simulink model "DWPT_fixed"  (R2026b)
settings: Solver=ode3  StopTime=0.07  FixedStep=Ts  MaxStep=1.0E-7  RelTol=1e-4  AbsTol=1e-6
model workspace (MAT data in the model file):
  CP1 = 9.03e-09
  CP2 = 9.23e-09
  CS = 1.25e-08
  CT1 = 5.5e-08
  CT2 = 5.4e-08
  Fs = 34000000
  LP1 = 0.0004373
  LP2 = 0.0004206
  LS = 0.000306
  LT1 = 9.8e-05
  LT2 = 9.95e-05
  M1 = 9.4e-05
  M2 = 0
  RL = 30
  RP1 = 1.4
  RP2 = 1.4
  RS = 1.3
  Ts = 2.94117647059e-08
  Vdc = 50
  averageCycles = 100
  f = 85000
  samplesPerPeriod = 400
undefined symbols (not defined in the file or in its folder): ee_sli_rtmsupport, G, gcbh
libraries: sl_signal_attributes x63, eeGeneralControl x40, fl_lib x32, nesl_utility x23, eeGeneralMeasurement x14, ee_lib x9, dspfdesign x1
(part 3 of 3)

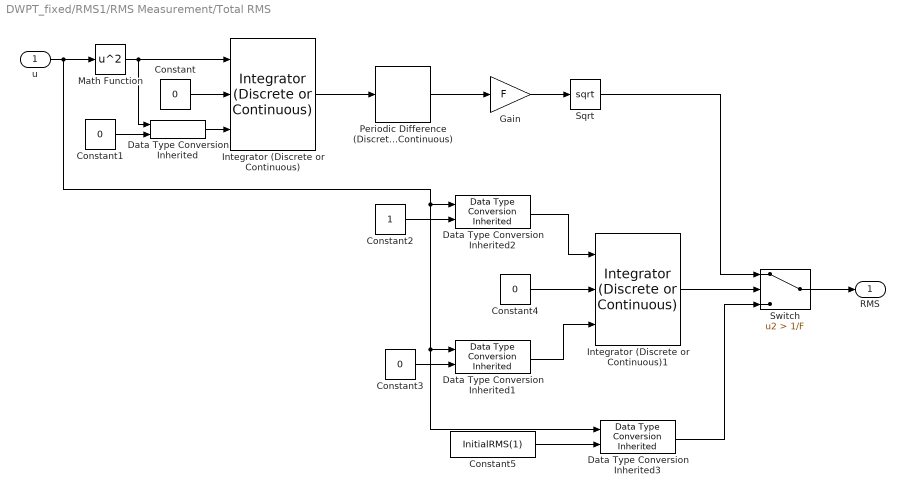
== system DWPT_fixed/RMS1/RMS Measurement/Total RMS ==
  u : Inport
  Constant{,1,3..4} (4 alike) : Constant  Value=0
  Constant2 : Constant
  Constant5 : Constant  Value=InitialRMS(1)
  Data Type Conversion Inherited{,1..3} (4 alike) : sl_signal_attributes/Data Type Conversion Inherited  ConvertRealWorld=Real World Value  DoSatur=off
  Gain : Gain  Gain=F
  Integrator (Discrete or Continuous) : eeGeneralControl/Integrator (Discrete or Continuous)  LabelModeActiveChoice=Continuous  IntegratorMethod=Integration: Forward Euler  ExternalReset=level  LimitType=Anti-windup  B=inf  A=-inf  Ts=Ts
  Integrator (Discrete or Continuous)1 : eeGeneralControl/Integrator (Discrete or Continuous)  LabelModeActiveChoice=Continuous  IntegratorMethod=Integration: Forward Euler  ExternalReset=level  LimitType=Anti-windup  B=2/F  A=-inf  Ts=Ts
  Math Function : Math  Operator=square  SignedPower=on
  Periodic Difference (Discrete or Continuous) : eeGeneralMeasurement/Periodic Difference (Discrete or Continuous)  LabelModeActiveChoice=Continuous  F=F  Ts=Ts
      link override Continuous/Transport Delay: BufferSize=262144
  Sqrt : Sqrt
  Switch : Switch  Criteria=u2 > Threshold  Threshold=1/F  SaturateOnIntegerOverflow=off  InputSameDT=off
  RMS : Outport  VectorParamsAs1DForOutWhenUnconnected=off
  wires:
  Sqrt/1 -> Switch/1
  Switch/1 -> RMS/1
  Constant2/1 -> Data Type Conversion Inherited2/2
  Constant3/1 -> Data Type Conversion Inherited1/2
  Constant4/1 -> Integrator (Discrete or Continuous)1/2
  Data Type Conversion Inherited3/1 -> Switch/3
  Constant5/1 -> Data Type Conversion Inherited3/2
  Data Type Conversion Inherited2/1 -> Integrator (Discrete or Continuous)1/1
  Data Type Conversion Inherited1/1 -> Integrator (Discrete or Continuous)1/3
  Integrator (Discrete or Continuous)1/1 -> Switch/2
  Constant1/1 -> Data Type Conversion Inherited/2
  Data Type Conversion Inherited/1 -> Integrator (Discrete or Continuous)/3
  Periodic Difference (Discrete or Continuous)/1 -> Gain/1
  Gain/1 -> Sqrt/1
  Integrator (Discrete or Continuous)/1 -> Periodic Difference (Discrete or Continuous)/1
  u/1 -> Math Function/1, Data Type Conversion Inherited2/1, Data Type Conversion Inherited3/1, Data Type Conversion Inherited1/1
  Math Function/1 -> Integrator (Discrete or Continuous)/1, Data Type Conversion Inherited/1
  Constant/1 -> Integrator (Discrete or Continuous)/2

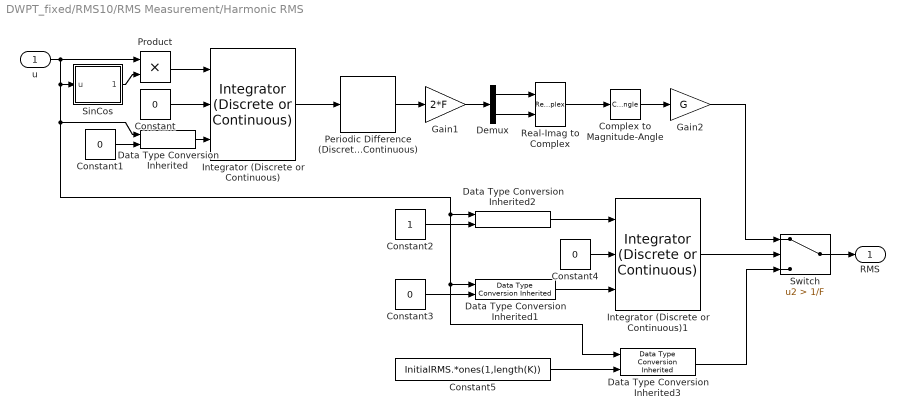
== system DWPT_fixed/RMS10/RMS Measurement/Harmonic RMS ==
  u : Inport
  Complex to Magnitude-Angle : ComplexToMagnitudeAngle  Output=Magnitude
  Constant{,1,3..4} (4 alike) : Constant  Value=0
  Constant2 : Constant
  Constant5 : Constant  Value=InitialRMS.*ones(1,length(K))
  Data Type Conversion Inherited{,1..3} (4 alike) : sl_signal_attributes/Data Type Conversion Inherited  ConvertRealWorld=Real World Value  DoSatur=off
  Demux : Demux  Outputs=2
  Gain1 : Gain  Gain=2*F
  Gain2 : Gain  Gain=G
  Integrator (Discrete or Continuous) : eeGeneralControl/Integrator (Discrete or Continuous)  LabelModeActiveChoice=Continuous  IntegratorMethod=Integration: Forward Euler  ExternalReset=level  LimitType=Anti-windup  B=inf  A=-inf  Ts=Ts
  Integrator (Discrete or Continuous)1 : eeGeneralControl/Integrator (Discrete or Continuous)  LabelModeActiveChoice=Continuous  IntegratorMethod=Integration: Forward Euler  ExternalReset=level  LimitType=Anti-windup  B=2/F  A=-inf  Ts=Ts
  Periodic Difference (Discrete or Continuous) : eeGeneralMeasurement/Periodic Difference (Discrete or Continuous)  LabelModeActiveChoice=Continuous  F=F  Ts=Ts
      link override Continuous/Transport Delay: BufferSize=262144
  Product : Product
  Real-Imag to Complex : RealImagToComplex
  SinCos : Subsystem
  Switch : Switch  Criteria=u2 > Threshold  Threshold=1/F  SaturateOnIntegerOverflow=off  InputSameDT=off
  RMS : Outport  VectorParamsAs1DForOutWhenUnconnected=off
  wires:
  Switch/1 -> RMS/1
  Gain2/1 -> Switch/1
  Constant2/1 -> Data Type Conversion Inherited2/2
  Constant3/1 -> Data Type Conversion Inherited1/2
  Constant4/1 -> Integrator (Discrete or Continuous)1/2
  Data Type Conversion Inherited3/1 -> Switch/3
  Constant5/1 -> Data Type Conversion Inherited3/2
  Data Type Conversion Inherited2/1 -> Integrator (Discrete or Continuous)1/1
  Data Type Conversion Inherited1/1 -> Integrator (Discrete or Continuous)1/3
  Integrator (Discrete or Continuous)1/1 -> Switch/2
  Constant1/1 -> Data Type Conversion Inherited/2
  Data Type Conversion Inherited/1 -> Integrator (Discrete or Continuous)/3
  Integrator (Discrete or Continuous)/1 -> Periodic Difference (Discrete or Continuous)/1
  Constant/1 -> Integrator (Discrete or Continuous)/2
  Demux/2 -> Real-Imag to Complex/2
  u/1 -> SinCos/1(u), Data Type Conversion Inherited/1, Data Type Conversion Inherited2/1, Data Type Conversion Inherited1/1, Data Type Conversion Inherited3/1, Product/1
  Periodic Difference (Discrete or Continuous)/1 -> Gain1/1
  Real-Imag to Complex/1 -> Complex to Magnitude-Angle/1
  Demux/1 -> Real-Imag to Complex/1
  SinCos/1(SinCos) -> Product/2
  Gain1/1 -> Demux/1
  Product/1 -> Integrator (Discrete or Continuous)/1
  Complex to Magnitude-Angle/1 -> Gain2/1

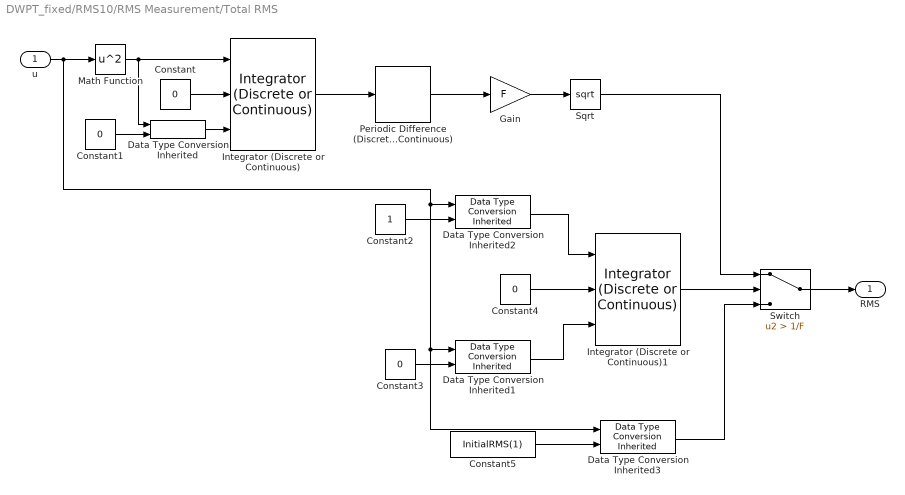
== system DWPT_fixed/RMS10/RMS Measurement/Total RMS ==
  u : Inport
  Constant{,1,3..4} (4 alike) : Constant  Value=0
  Constant2 : Constant
  Constant5 : Constant  Value=InitialRMS(1)
  Data Type Conversion Inherited{,1..3} (4 alike) : sl_signal_attributes/Data Type Conversion Inherited  ConvertRealWorld=Real World Value  DoSatur=off
  Gain : Gain  Gain=F
  Integrator (Discrete or Continuous) : eeGeneralControl/Integrator (Discrete or Continuous)  LabelModeActiveChoice=Continuous  IntegratorMethod=Integration: Forward Euler  ExternalReset=level  LimitType=Anti-windup  B=inf  A=-inf  Ts=Ts
  Integrator (Discrete or Continuous)1 : eeGeneralControl/Integrator (Discrete or Continuous)  LabelModeActiveChoice=Continuous  IntegratorMethod=Integration: Forward Euler  ExternalReset=level  LimitType=Anti-windup  B=2/F  A=-inf  Ts=Ts
  Math Function : Math  Operator=square  SignedPower=on
  Periodic Difference (Discrete or Continuous) : eeGeneralMeasurement/Periodic Difference (Discrete or Continuous)  LabelModeActiveChoice=Continuous  F=F  Ts=Ts
      link override Continuous/Transport Delay: BufferSize=262144
  Sqrt : Sqrt
  Switch : Switch  Criteria=u2 > Threshold  Threshold=1/F  SaturateOnIntegerOverflow=off  InputSameDT=off
  RMS : Outport  VectorParamsAs1DForOutWhenUnconnected=off
  wires:
  Sqrt/1 -> Switch/1
  Switch/1 -> RMS/1
  Constant2/1 -> Data Type Conversion Inherited2/2
  Constant3/1 -> Data Type Conversion Inherited1/2
  Constant4/1 -> Integrator (Discrete or Continuous)1/2
  Data Type Conversion Inherited3/1 -> Switch/3
  Constant5/1 -> Data Type Conversion Inherited3/2
  Data Type Conversion Inherited2/1 -> Integrator (Discrete or Continuous)1/1
  Data Type Conversion Inherited1/1 -> Integrator (Discrete or Continuous)1/3
  Integrator (Discrete or Continuous)1/1 -> Switch/2
  Constant1/1 -> Data Type Conversion Inherited/2
  Data Type Conversion Inherited/1 -> Integrator (Discrete or Continuous)/3
  Periodic Difference (Discrete or Continuous)/1 -> Gain/1
  Gain/1 -> Sqrt/1
  Integrator (Discrete or Continuous)/1 -> Periodic Difference (Discrete or Continuous)/1
  u/1 -> Math Function/1, Data Type Conversion Inherited2/1, Data Type Conversion Inherited3/1, Data Type Conversion Inherited1/1
  Math Function/1 -> Integrator (Discrete or Continuous)/1, Data Type Conversion Inherited/1
  Constant/1 -> Integrator (Discrete or Continuous)/2

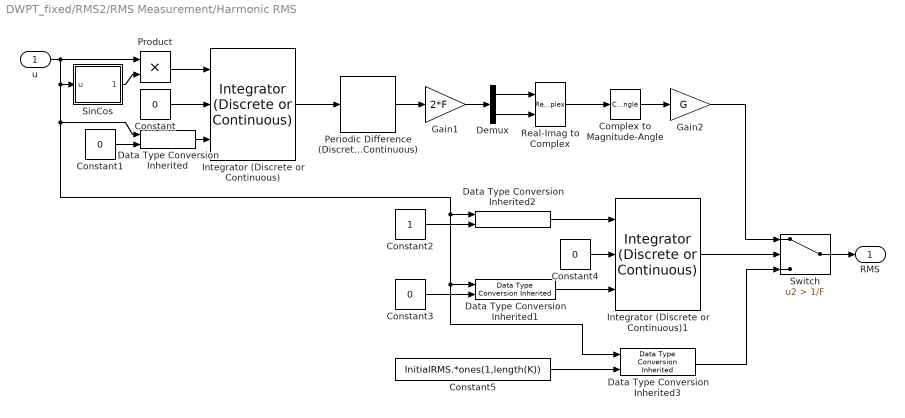
== system DWPT_fixed/RMS2/RMS Measurement/Harmonic RMS ==
  u : Inport
  Complex to Magnitude-Angle : ComplexToMagnitudeAngle  Output=Magnitude
  Constant{,1,3..4} (4 alike) : Constant  Value=0
  Constant2 : Constant
  Constant5 : Constant  Value=InitialRMS.*ones(1,length(K))
  Data Type Conversion Inherited{,1..3} (4 alike) : sl_signal_attributes/Data Type Conversion Inherited  ConvertRealWorld=Real World Value  DoSatur=off
  Demux : Demux  Outputs=2
  Gain1 : Gain  Gain=2*F
  Gain2 : Gain  Gain=G
  Integrator (Discrete or Continuous) : eeGeneralControl/Integrator (Discrete or Continuous)  LabelModeActiveChoice=Continuous  IntegratorMethod=Integration: Forward Euler  ExternalReset=level  LimitType=Anti-windup  B=inf  A=-inf  Ts=Ts
  Integrator (Discrete or Continuous)1 : eeGeneralControl/Integrator (Discrete or Continuous)  LabelModeActiveChoice=Continuous  IntegratorMethod=Integration: Forward Euler  ExternalReset=level  LimitType=Anti-windup  B=2/F  A=-inf  Ts=Ts
  Periodic Difference (Discrete or Continuous) : eeGeneralMeasurement/Periodic Difference (Discrete or Continuous)  LabelModeActiveChoice=Continuous  F=F  Ts=Ts
      link override Continuous/Transport Delay: BufferSize=262144
  Product : Product
  Real-Imag to Complex : RealImagToComplex
  SinCos : Subsystem
  Switch : Switch  Criteria=u2 > Threshold  Threshold=1/F  SaturateOnIntegerOverflow=off  InputSameDT=off
  RMS : Outport  VectorParamsAs1DForOutWhenUnconnected=off
  wires:
  Switch/1 -> RMS/1
  Gain2/1 -> Switch/1
  Constant2/1 -> Data Type Conversion Inherited2/2
  Constant3/1 -> Data Type Conversion Inherited1/2
  Constant4/1 -> Integrator (Discrete or Continuous)1/2
  Data Type Conversion Inherited3/1 -> Switch/3
  Constant5/1 -> Data Type Conversion Inherited3/2
  Data Type Conversion Inherited2/1 -> Integrator (Discrete or Continuous)1/1
  Data Type Conversion Inherited1/1 -> Integrator (Discrete or Continuous)1/3
  Integrator (Discrete or Continuous)1/1 -> Switch/2
  Constant1/1 -> Data Type Conversion Inherited/2
  Data Type Conversion Inherited/1 -> Integrator (Discrete or Continuous)/3
  Integrator (Discrete or Continuous)/1 -> Periodic Difference (Discrete or Continuous)/1
  Constant/1 -> Integrator (Discrete or Continuous)/2
  Demux/2 -> Real-Imag to Complex/2
  u/1 -> SinCos/1(u), Data Type Conversion Inherited/1, Data Type Conversion Inherited2/1, Data Type Conversion Inherited1/1, Data Type Conversion Inherited3/1, Product/1
  Periodic Difference (Discrete or Continuous)/1 -> Gain1/1
  Real-Imag to Complex/1 -> Complex to Magnitude-Angle/1
  Demux/1 -> Real-Imag to Complex/1
  SinCos/1(SinCos) -> Product/2
  Gain1/1 -> Demux/1
  Product/1 -> Integrator (Discrete or Continuous)/1
  Complex to Magnitude-Angle/1 -> Gain2/1

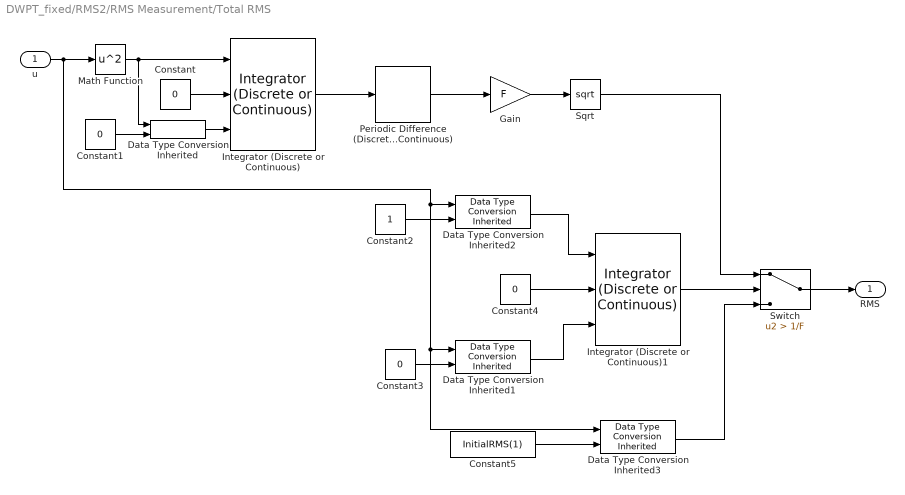
== system DWPT_fixed/RMS2/RMS Measurement/Total RMS ==
  u : Inport
  Constant{,1,3..4} (4 alike) : Constant  Value=0
  Constant2 : Constant
  Constant5 : Constant  Value=InitialRMS(1)
  Data Type Conversion Inherited{,1..3} (4 alike) : sl_signal_attributes/Data Type Conversion Inherited  ConvertRealWorld=Real World Value  DoSatur=off
  Gain : Gain  Gain=F
  Integrator (Discrete or Continuous) : eeGeneralControl/Integrator (Discrete or Continuous)  LabelModeActiveChoice=Continuous  IntegratorMethod=Integration: Forward Euler  ExternalReset=level  LimitType=Anti-windup  B=inf  A=-inf  Ts=Ts
  Integrator (Discrete or Continuous)1 : eeGeneralControl/Integrator (Discrete or Continuous)  LabelModeActiveChoice=Continuous  IntegratorMethod=Integration: Forward Euler  ExternalReset=level  LimitType=Anti-windup  B=2/F  A=-inf  Ts=Ts
  Math Function : Math  Operator=square  SignedPower=on
  Periodic Difference (Discrete or Continuous) : eeGeneralMeasurement/Periodic Difference (Discrete or Continuous)  LabelModeActiveChoice=Continuous  F=F  Ts=Ts
      link override Continuous/Transport Delay: BufferSize=262144
  Sqrt : Sqrt
  Switch : Switch  Criteria=u2 > Threshold  Threshold=1/F  SaturateOnIntegerOverflow=off  InputSameDT=off
  RMS : Outport  VectorParamsAs1DForOutWhenUnconnected=off
  wires:
  Sqrt/1 -> Switch/1
  Switch/1 -> RMS/1
  Constant2/1 -> Data Type Conversion Inherited2/2
  Constant3/1 -> Data Type Conversion Inherited1/2
  Constant4/1 -> Integrator (Discrete or Continuous)1/2
  Data Type Conversion Inherited3/1 -> Switch/3
  Constant5/1 -> Data Type Conversion Inherited3/2
  Data Type Conversion Inherited2/1 -> Integrator (Discrete or Continuous)1/1
  Data Type Conversion Inherited1/1 -> Integrator (Discrete or Continuous)1/3
  Integrator (Discrete or Continuous)1/1 -> Switch/2
  Constant1/1 -> Data Type Conversion Inherited/2
  Data Type Conversion Inherited/1 -> Integrator (Discrete or Continuous)/3
  Periodic Difference (Discrete or Continuous)/1 -> Gain/1
  Gain/1 -> Sqrt/1
  Integrator (Discrete or Continuous)/1 -> Periodic Difference (Discrete or Continuous)/1
  u/1 -> Math Function/1, Data Type Conversion Inherited2/1, Data Type Conversion Inherited3/1, Data Type Conversion Inherited1/1
  Math Function/1 -> Integrator (Discrete or Continuous)/1, Data Type Conversion Inherited/1
  Constant/1 -> Integrator (Discrete or Continuous)/2

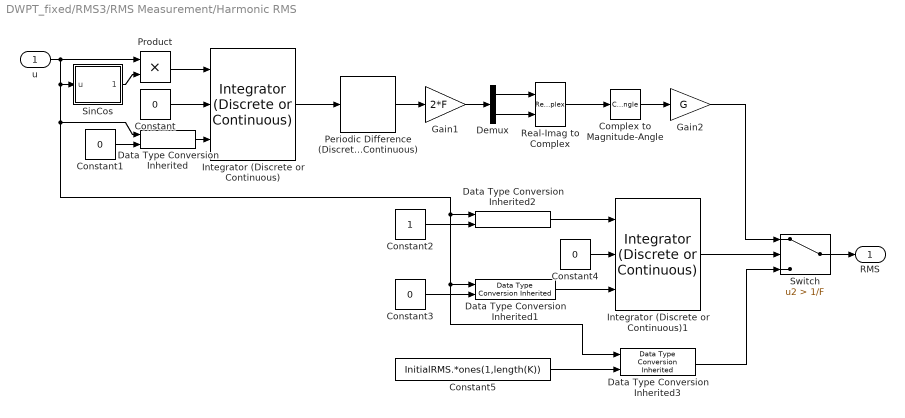
== system DWPT_fixed/RMS3/RMS Measurement/Harmonic RMS ==
  u : Inport
  Complex to Magnitude-Angle : ComplexToMagnitudeAngle  Output=Magnitude
  Constant{,1,3..4} (4 alike) : Constant  Value=0
  Constant2 : Constant
  Constant5 : Constant  Value=InitialRMS.*ones(1,length(K))
  Data Type Conversion Inherited{,1..3} (4 alike) : sl_signal_attributes/Data Type Conversion Inherited  ConvertRealWorld=Real World Value  DoSatur=off
  Demux : Demux  Outputs=2
  Gain1 : Gain  Gain=2*F
  Gain2 : Gain  Gain=G
  Integrator (Discrete or Continuous) : eeGeneralControl/Integrator (Discrete or Continuous)  LabelModeActiveChoice=Continuous  IntegratorMethod=Integration: Forward Euler  ExternalReset=level  LimitType=Anti-windup  B=inf  A=-inf  Ts=Ts
  Integrator (Discrete or Continuous)1 : eeGeneralControl/Integrator (Discrete or Continuous)  LabelModeActiveChoice=Continuous  IntegratorMethod=Integration: Forward Euler  ExternalReset=level  LimitType=Anti-windup  B=2/F  A=-inf  Ts=Ts
  Periodic Difference (Discrete or Continuous) : eeGeneralMeasurement/Periodic Difference (Discrete or Continuous)  LabelModeActiveChoice=Continuous  F=F  Ts=Ts
      link override Continuous/Transport Delay: BufferSize=262144
  Product : Product
  Real-Imag to Complex : RealImagToComplex
  SinCos : Subsystem
  Switch : Switch  Criteria=u2 > Threshold  Threshold=1/F  SaturateOnIntegerOverflow=off  InputSameDT=off
  RMS : Outport  VectorParamsAs1DForOutWhenUnconnected=off
  wires:
  Switch/1 -> RMS/1
  Gain2/1 -> Switch/1
  Constant2/1 -> Data Type Conversion Inherited2/2
  Constant3/1 -> Data Type Conversion Inherited1/2
  Constant4/1 -> Integrator (Discrete or Continuous)1/2
  Data Type Conversion Inherited3/1 -> Switch/3
  Constant5/1 -> Data Type Conversion Inherited3/2
  Data Type Conversion Inherited2/1 -> Integrator (Discrete or Continuous)1/1
  Data Type Conversion Inherited1/1 -> Integrator (Discrete or Continuous)1/3
  Integrator (Discrete or Continuous)1/1 -> Switch/2
  Constant1/1 -> Data Type Conversion Inherited/2
  Data Type Conversion Inherited/1 -> Integrator (Discrete or Continuous)/3
  Integrator (Discrete or Continuous)/1 -> Periodic Difference (Discrete or Continuous)/1
  Constant/1 -> Integrator (Discrete or Continuous)/2
  Demux/2 -> Real-Imag to Complex/2
  u/1 -> SinCos/1(u), Data Type Conversion Inherited/1, Data Type Conversion Inherited2/1, Data Type Conversion Inherited1/1, Data Type Conversion Inherited3/1, Product/1
  Periodic Difference (Discrete or Continuous)/1 -> Gain1/1
  Real-Imag to Complex/1 -> Complex to Magnitude-Angle/1
  Demux/1 -> Real-Imag to Complex/1
  SinCos/1(SinCos) -> Product/2
  Gain1/1 -> Demux/1
  Product/1 -> Integrator (Discrete or Continuous)/1
  Complex to Magnitude-Angle/1 -> Gain2/1

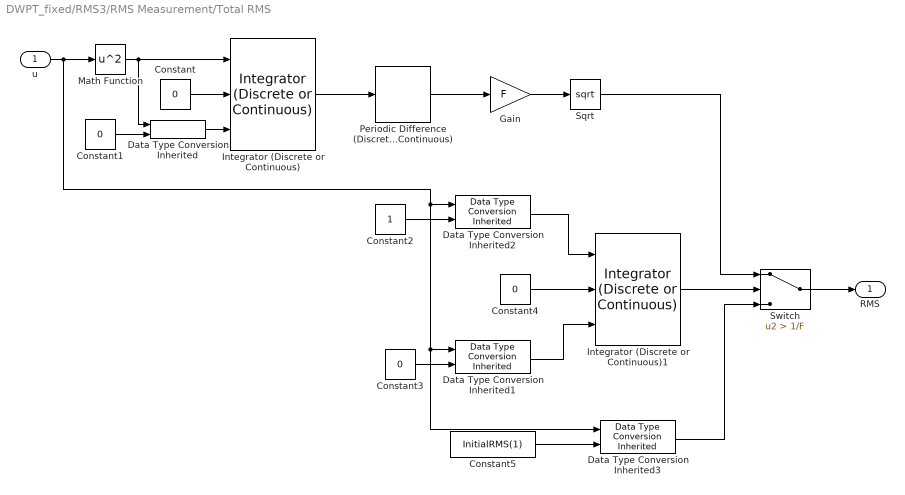
== system DWPT_fixed/RMS3/RMS Measurement/Total RMS ==
  u : Inport
  Constant{,1,3..4} (4 alike) : Constant  Value=0
  Constant2 : Constant
  Constant5 : Constant  Value=InitialRMS(1)
  Data Type Conversion Inherited{,1..3} (4 alike) : sl_signal_attributes/Data Type Conversion Inherited  ConvertRealWorld=Real World Value  DoSatur=off
  Gain : Gain  Gain=F
  Integrator (Discrete or Continuous) : eeGeneralControl/Integrator (Discrete or Continuous)  LabelModeActiveChoice=Continuous  IntegratorMethod=Integration: Forward Euler  ExternalReset=level  LimitType=Anti-windup  B=inf  A=-inf  Ts=Ts
  Integrator (Discrete or Continuous)1 : eeGeneralControl/Integrator (Discrete or Continuous)  LabelModeActiveChoice=Continuous  IntegratorMethod=Integration: Forward Euler  ExternalReset=level  LimitType=Anti-windup  B=2/F  A=-inf  Ts=Ts
  Math Function : Math  Operator=square  SignedPower=on
  Periodic Difference (Discrete or Continuous) : eeGeneralMeasurement/Periodic Difference (Discrete or Continuous)  LabelModeActiveChoice=Continuous  F=F  Ts=Ts
      link override Continuous/Transport Delay: BufferSize=262144
  Sqrt : Sqrt
  Switch : Switch  Criteria=u2 > Threshold  Threshold=1/F  SaturateOnIntegerOverflow=off  InputSameDT=off
  RMS : Outport  VectorParamsAs1DForOutWhenUnconnected=off
  wires:
  Sqrt/1 -> Switch/1
  Switch/1 -> RMS/1
  Constant2/1 -> Data Type Conversion Inherited2/2
  Constant3/1 -> Data Type Conversion Inherited1/2
  Constant4/1 -> Integrator (Discrete or Continuous)1/2
  Data Type Conversion Inherited3/1 -> Switch/3
  Constant5/1 -> Data Type Conversion Inherited3/2
  Data Type Conversion Inherited2/1 -> Integrator (Discrete or Continuous)1/1
  Data Type Conversion Inherited1/1 -> Integrator (Discrete or Continuous)1/3
  Integrator (Discrete or Continuous)1/1 -> Switch/2
  Constant1/1 -> Data Type Conversion Inherited/2
  Data Type Conversion Inherited/1 -> Integrator (Discrete or Continuous)/3
  Periodic Difference (Discrete or Continuous)/1 -> Gain/1
  Gain/1 -> Sqrt/1
  Integrator (Discrete or Continuous)/1 -> Periodic Difference (Discrete or Continuous)/1
  u/1 -> Math Function/1, Data Type Conversion Inherited2/1, Data Type Conversion Inherited3/1, Data Type Conversion Inherited1/1
  Math Function/1 -> Integrator (Discrete or Continuous)/1, Data Type Conversion Inherited/1
  Constant/1 -> Integrator (Discrete or Continuous)/2

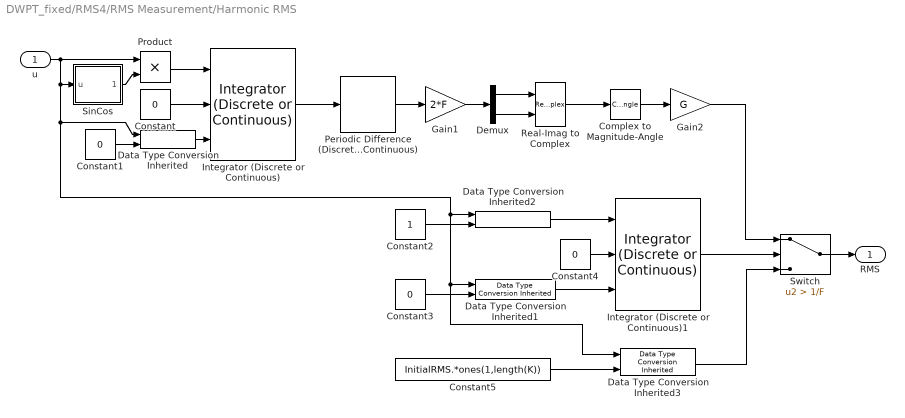
== system DWPT_fixed/RMS4/RMS Measurement/Harmonic RMS ==
  u : Inport
  Complex to Magnitude-Angle : ComplexToMagnitudeAngle  Output=Magnitude
  Constant{,1,3..4} (4 alike) : Constant  Value=0
  Constant2 : Constant
  Constant5 : Constant  Value=InitialRMS.*ones(1,length(K))
  Data Type Conversion Inherited{,1..3} (4 alike) : sl_signal_attributes/Data Type Conversion Inherited  ConvertRealWorld=Real World Value  DoSatur=off
  Demux : Demux  Outputs=2
  Gain1 : Gain  Gain=2*F
  Gain2 : Gain  Gain=G
  Integrator (Discrete or Continuous) : eeGeneralControl/Integrator (Discrete or Continuous)  LabelModeActiveChoice=Continuous  IntegratorMethod=Integration: Forward Euler  ExternalReset=level  LimitType=Anti-windup  B=inf  A=-inf  Ts=Ts
  Integrator (Discrete or Continuous)1 : eeGeneralControl/Integrator (Discrete or Continuous)  LabelModeActiveChoice=Continuous  IntegratorMethod=Integration: Forward Euler  ExternalReset=level  LimitType=Anti-windup  B=2/F  A=-inf  Ts=Ts
  Periodic Difference (Discrete or Continuous) : eeGeneralMeasurement/Periodic Difference (Discrete or Continuous)  LabelModeActiveChoice=Continuous  F=F  Ts=Ts
      link override Continuous/Transport Delay: BufferSize=262144
  Product : Product
  Real-Imag to Complex : RealImagToComplex
  SinCos : Subsystem
  Switch : Switch  Criteria=u2 > Threshold  Threshold=1/F  SaturateOnIntegerOverflow=off  InputSameDT=off
  RMS : Outport  VectorParamsAs1DForOutWhenUnconnected=off
  wires:
  Switch/1 -> RMS/1
  Gain2/1 -> Switch/1
  Constant2/1 -> Data Type Conversion Inherited2/2
  Constant3/1 -> Data Type Conversion Inherited1/2
  Constant4/1 -> Integrator (Discrete or Continuous)1/2
  Data Type Conversion Inherited3/1 -> Switch/3
  Constant5/1 -> Data Type Conversion Inherited3/2
  Data Type Conversion Inherited2/1 -> Integrator (Discrete or Continuous)1/1
  Data Type Conversion Inherited1/1 -> Integrator (Discrete or Continuous)1/3
  Integrator (Discrete or Continuous)1/1 -> Switch/2
  Constant1/1 -> Data Type Conversion Inherited/2
  Data Type Conversion Inherited/1 -> Integrator (Discrete or Continuous)/3
  Integrator (Discrete or Continuous)/1 -> Periodic Difference (Discrete or Continuous)/1
  Constant/1 -> Integrator (Discrete or Continuous)/2
  Demux/2 -> Real-Imag to Complex/2
  u/1 -> SinCos/1(u), Data Type Conversion Inherited/1, Data Type Conversion Inherited2/1, Data Type Conversion Inherited1/1, Data Type Conversion Inherited3/1, Product/1
  Periodic Difference (Discrete or Continuous)/1 -> Gain1/1
  Real-Imag to Complex/1 -> Complex to Magnitude-Angle/1
  Demux/1 -> Real-Imag to Complex/1
  SinCos/1(SinCos) -> Product/2
  Gain1/1 -> Demux/1
  Product/1 -> Integrator (Discrete or Continuous)/1
  Complex to Magnitude-Angle/1 -> Gain2/1

== system DWPT_fixed/RMS4/RMS Measurement/Total RMS ==
  u : Inport
  Constant{,1,3..4} (4 alike) : Constant  Value=0
  Constant2 : Constant
  Constant5 : Constant  Value=InitialRMS(1)
  Data Type Conversion Inherited{,1..3} (4 alike) : sl_signal_attributes/Data Type Conversion Inherited  ConvertRealWorld=Real World Value  DoSatur=off
  Gain : Gain  Gain=F
  Integrator (Discrete or Continuous) : eeGeneralControl/Integrator (Discrete or Continuous)  LabelModeActiveChoice=Continuous  IntegratorMethod=Integration: Forward Euler  ExternalReset=level  LimitType=Anti-windup  B=inf  A=-inf  Ts=Ts
  Integrator (Discrete or Continuous)1 : eeGeneralControl/Integrator (Discrete or Continuous)  LabelModeActiveChoice=Continuous  IntegratorMethod=Integration: Forward Euler  ExternalReset=level  LimitType=Anti-windup  B=2/F  A=-inf  Ts=Ts
  Math Function : Math  Operator=square  SignedPower=on
  Periodic Difference (Discrete or Continuous) : eeGeneralMeasurement/Periodic Difference (Discrete or Continuous)  LabelModeActiveChoice=Continuous  F=F  Ts=Ts
      link override Continuous/Transport Delay: BufferSize=262144
  Sqrt : Sqrt
  Switch : Switch  Criteria=u2 > Threshold  Threshold=1/F  SaturateOnIntegerOverflow=off  InputSameDT=off
  RMS : Outport  VectorParamsAs1DForOutWhenUnconnected=off
  wires:
  Sqrt/1 -> Switch/1
  Switch/1 -> RMS/1
  Constant2/1 -> Data Type Conversion Inherited2/2
  Constant3/1 -> Data Type Conversion Inherited1/2
  Constant4/1 -> Integrator (Discrete or Continuous)1/2
  Data Type Conversion Inherited3/1 -> Switch/3
  Constant5/1 -> Data Type Conversion Inherited3/2
  Data Type Conversion Inherited2/1 -> Integrator (Discrete or Continuous)1/1
  Data Type Conversion Inherited1/1 -> Integrator (Discrete or Continuous)1/3
  Integrator (Discrete or Continuous)1/1 -> Switch/2
  Constant1/1 -> Data Type Conversion Inherited/2
  Data Type Conversion Inherited/1 -> Integrator (Discrete or Continuous)/3
  Periodic Difference (Discrete or Continuous)/1 -> Gain/1
  Gain/1 -> Sqrt/1
  Integrator (Discrete or Continuous)/1 -> Periodic Difference (Discrete or Continuous)/1
  u/1 -> Math Function/1, Data Type Conversion Inherited2/1, Data Type Conversion Inherited3/1, Data Type Conversion Inherited1/1
  Math Function/1 -> Integrator (Discrete or Continuous)/1, Data Type Conversion Inherited/1
  Constant/1 -> Integrator (Discrete or Continuous)/2

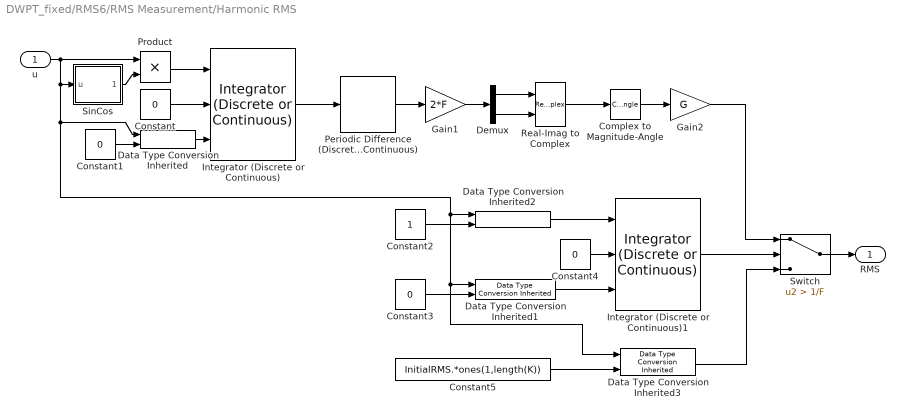
== system DWPT_fixed/RMS6/RMS Measurement/Harmonic RMS ==
  u : Inport
  Complex to Magnitude-Angle : ComplexToMagnitudeAngle  Output=Magnitude
  Constant{,1,3..4} (4 alike) : Constant  Value=0
  Constant2 : Constant
  Constant5 : Constant  Value=InitialRMS.*ones(1,length(K))
  Data Type Conversion Inherited{,1..3} (4 alike) : sl_signal_attributes/Data Type Conversion Inherited  ConvertRealWorld=Real World Value  DoSatur=off
  Demux : Demux  Outputs=2
  Gain1 : Gain  Gain=2*F
  Gain2 : Gain  Gain=G
  Integrator (Discrete or Continuous) : eeGeneralControl/Integrator (Discrete or Continuous)  LabelModeActiveChoice=Continuous  IntegratorMethod=Integration: Forward Euler  ExternalReset=level  LimitType=Anti-windup  B=inf  A=-inf  Ts=Ts
  Integrator (Discrete or Continuous)1 : eeGeneralControl/Integrator (Discrete or Continuous)  LabelModeActiveChoice=Continuous  IntegratorMethod=Integration: Forward Euler  ExternalReset=level  LimitType=Anti-windup  B=2/F  A=-inf  Ts=Ts
  Periodic Difference (Discrete or Continuous) : eeGeneralMeasurement/Periodic Difference (Discrete or Continuous)  LabelModeActiveChoice=Continuous  F=F  Ts=Ts
      link override Continuous/Transport Delay: BufferSize=262144
  Product : Product
  Real-Imag to Complex : RealImagToComplex
  SinCos : Subsystem
  Switch : Switch  Criteria=u2 > Threshold  Threshold=1/F  SaturateOnIntegerOverflow=off  InputSameDT=off
  RMS : Outport  VectorParamsAs1DForOutWhenUnconnected=off
  wires:
  Switch/1 -> RMS/1
  Gain2/1 -> Switch/1
  Constant2/1 -> Data Type Conversion Inherited2/2
  Constant3/1 -> Data Type Conversion Inherited1/2
  Constant4/1 -> Integrator (Discrete or Continuous)1/2
  Data Type Conversion Inherited3/1 -> Switch/3
  Constant5/1 -> Data Type Conversion Inherited3/2
  Data Type Conversion Inherited2/1 -> Integrator (Discrete or Continuous)1/1
  Data Type Conversion Inherited1/1 -> Integrator (Discrete or Continuous)1/3
  Integrator (Discrete or Continuous)1/1 -> Switch/2
  Constant1/1 -> Data Type Conversion Inherited/2
  Data Type Conversion Inherited/1 -> Integrator (Discrete or Continuous)/3
  Integrator (Discrete or Continuous)/1 -> Periodic Difference (Discrete or Continuous)/1
  Constant/1 -> Integrator (Discrete or Continuous)/2
  Demux/2 -> Real-Imag to Complex/2
  u/1 -> SinCos/1(u), Data Type Conversion Inherited/1, Data Type Conversion Inherited2/1, Data Type Conversion Inherited1/1, Data Type Conversion Inherited3/1, Product/1
  Periodic Difference (Discrete or Continuous)/1 -> Gain1/1
  Real-Imag to Complex/1 -> Complex to Magnitude-Angle/1
  Demux/1 -> Real-Imag to Complex/1
  SinCos/1(SinCos) -> Product/2
  Gain1/1 -> Demux/1
  Product/1 -> Integrator (Discrete or Continuous)/1
  Complex to Magnitude-Angle/1 -> Gain2/1

== system DWPT_fixed/RMS6/RMS Measurement/Total RMS ==
  u : Inport
  Constant{,1,3..4} (4 alike) : Constant  Value=0
  Constant2 : Constant
  Constant5 : Constant  Value=InitialRMS(1)
  Data Type Conversion Inherited{,1..3} (4 alike) : sl_signal_attributes/Data Type Conversion Inherited  ConvertRealWorld=Real World Value  DoSatur=off
  Gain : Gain  Gain=F
  Integrator (Discrete or Continuous) : eeGeneralControl/Integrator (Discrete or Continuous)  LabelModeActiveChoice=Continuous  IntegratorMethod=Integration: Forward Euler  ExternalReset=level  LimitType=Anti-windup  B=inf  A=-inf  Ts=Ts
  Integrator (Discrete or Continuous)1 : eeGeneralControl/Integrator (Discrete or Continuous)  LabelModeActiveChoice=Continuous  IntegratorMethod=Integration: Forward Euler  ExternalReset=level  LimitType=Anti-windup  B=2/F  A=-inf  Ts=Ts
  Math Function : Math  Operator=square  SignedPower=on
  Periodic Difference (Discrete or Continuous) : eeGeneralMeasurement/Periodic Difference (Discrete or Continuous)  LabelModeActiveChoice=Continuous  F=F  Ts=Ts
      link override Continuous/Transport Delay: BufferSize=262144
  Sqrt : Sqrt
  Switch : Switch  Criteria=u2 > Threshold  Threshold=1/F  SaturateOnIntegerOverflow=off  InputSameDT=off
  RMS : Outport  VectorParamsAs1DForOutWhenUnconnected=off
  wires:
  Sqrt/1 -> Switch/1
  Switch/1 -> RMS/1
  Constant2/1 -> Data Type Conversion Inherited2/2
  Constant3/1 -> Data Type Conversion Inherited1/2
  Constant4/1 -> Integrator (Discrete or Continuous)1/2
  Data Type Conversion Inherited3/1 -> Switch/3
  Constant5/1 -> Data Type Conversion Inherited3/2
  Data Type Conversion Inherited2/1 -> Integrator (Discrete or Continuous)1/1
  Data Type Conversion Inherited1/1 -> Integrator (Discrete or Continuous)1/3
  Integrator (Discrete or Continuous)1/1 -> Switch/2
  Constant1/1 -> Data Type Conversion Inherited/2
  Data Type Conversion Inherited/1 -> Integrator (Discrete or Continuous)/3
  Periodic Difference (Discrete or Continuous)/1 -> Gain/1
  Gain/1 -> Sqrt/1
  Integrator (Discrete or Continuous)/1 -> Periodic Difference (Discrete or Continuous)/1
  u/1 -> Math Function/1, Data Type Conversion Inherited2/1, Data Type Conversion Inherited3/1, Data Type Conversion Inherited1/1
  Math Function/1 -> Integrator (Discrete or Continuous)/1, Data Type Conversion Inherited/1
  Constant/1 -> Integrator (Discrete or Continuous)/2

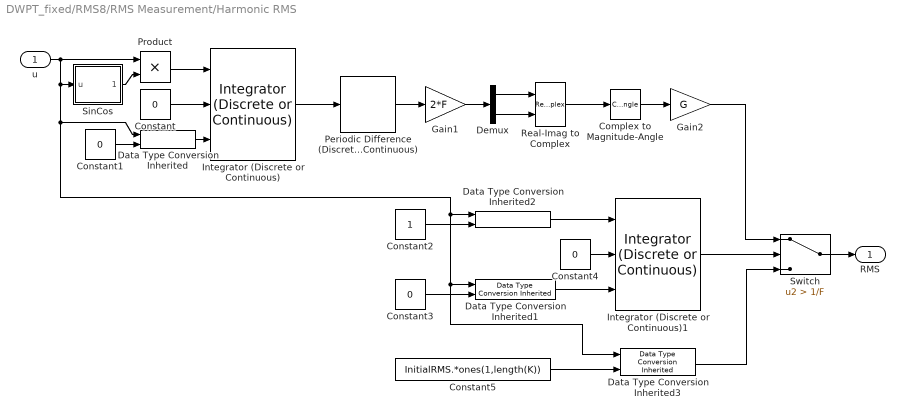
== system DWPT_fixed/RMS8/RMS Measurement/Harmonic RMS ==
  u : Inport
  Complex to Magnitude-Angle : ComplexToMagnitudeAngle  Output=Magnitude
  Constant{,1,3..4} (4 alike) : Constant  Value=0
  Constant2 : Constant
  Constant5 : Constant  Value=InitialRMS.*ones(1,length(K))
  Data Type Conversion Inherited{,1..3} (4 alike) : sl_signal_attributes/Data Type Conversion Inherited  ConvertRealWorld=Real World Value  DoSatur=off
  Demux : Demux  Outputs=2
  Gain1 : Gain  Gain=2*F
  Gain2 : Gain  Gain=G
  Integrator (Discrete or Continuous) : eeGeneralControl/Integrator (Discrete or Continuous)  LabelModeActiveChoice=Continuous  IntegratorMethod=Integration: Forward Euler  ExternalReset=level  LimitType=Anti-windup  B=inf  A=-inf  Ts=Ts
  Integrator (Discrete or Continuous)1 : eeGeneralControl/Integrator (Discrete or Continuous)  LabelModeActiveChoice=Continuous  IntegratorMethod=Integration: Forward Euler  ExternalReset=level  LimitType=Anti-windup  B=2/F  A=-inf  Ts=Ts
  Periodic Difference (Discrete or Continuous) : eeGeneralMeasurement/Periodic Difference (Discrete or Continuous)  LabelModeActiveChoice=Continuous  F=F  Ts=Ts
      link override Continuous/Transport Delay: BufferSize=262144
  Product : Product
  Real-Imag to Complex : RealImagToComplex
  SinCos : Subsystem
  Switch : Switch  Criteria=u2 > Threshold  Threshold=1/F  SaturateOnIntegerOverflow=off  InputSameDT=off
  RMS : Outport  VectorParamsAs1DForOutWhenUnconnected=off
  wires:
  Switch/1 -> RMS/1
  Gain2/1 -> Switch/1
  Constant2/1 -> Data Type Conversion Inherited2/2
  Constant3/1 -> Data Type Conversion Inherited1/2
  Constant4/1 -> Integrator (Discrete or Continuous)1/2
  Data Type Conversion Inherited3/1 -> Switch/3
  Constant5/1 -> Data Type Conversion Inherited3/2
  Data Type Conversion Inherited2/1 -> Integrator (Discrete or Continuous)1/1
  Data Type Conversion Inherited1/1 -> Integrator (Discrete or Continuous)1/3
  Integrator (Discrete or Continuous)1/1 -> Switch/2
  Constant1/1 -> Data Type Conversion Inherited/2
  Data Type Conversion Inherited/1 -> Integrator (Discrete or Continuous)/3
  Integrator (Discrete or Continuous)/1 -> Periodic Difference (Discrete or Continuous)/1
  Constant/1 -> Integrator (Discrete or Continuous)/2
  Demux/2 -> Real-Imag to Complex/2
  u/1 -> SinCos/1(u), Data Type Conversion Inherited/1, Data Type Conversion Inherited2/1, Data Type Conversion Inherited1/1, Data Type Conversion Inherited3/1, Product/1
  Periodic Difference (Discrete or Continuous)/1 -> Gain1/1
  Real-Imag to Complex/1 -> Complex to Magnitude-Angle/1
  Demux/1 -> Real-Imag to Complex/1
  SinCos/1(SinCos) -> Product/2
  Gain1/1 -> Demux/1
  Product/1 -> Integrator (Discrete or Continuous)/1
  Complex to Magnitude-Angle/1 -> Gain2/1

== system DWPT_fixed/RMS8/RMS Measurement/Total RMS ==
  u : Inport
  Constant{,1,3..4} (4 alike) : Constant  Value=0
  Constant2 : Constant
  Constant5 : Constant  Value=InitialRMS(1)
  Data Type Conversion Inherited{,1..3} (4 alike) : sl_signal_attributes/Data Type Conversion Inherited  ConvertRealWorld=Real World Value  DoSatur=off
  Gain : Gain  Gain=F
  Integrator (Discrete or Continuous) : eeGeneralControl/Integrator (Discrete or Continuous)  LabelModeActiveChoice=Continuous  IntegratorMethod=Integration: Forward Euler  ExternalReset=level  LimitType=Anti-windup  B=inf  A=-inf  Ts=Ts
  Integrator (Discrete or Continuous)1 : eeGeneralControl/Integrator (Discrete or Continuous)  LabelModeActiveChoice=Continuous  IntegratorMethod=Integration: Forward Euler  ExternalReset=level  LimitType=Anti-windup  B=2/F  A=-inf  Ts=Ts
  Math Function : Math  Operator=square  SignedPower=on
  Periodic Difference (Discrete or Continuous) : eeGeneralMeasurement/Periodic Difference (Discrete or Continuous)  LabelModeActiveChoice=Continuous  F=F  Ts=Ts
      link override Continuous/Transport Delay: BufferSize=262144
  Sqrt : Sqrt
  Switch : Switch  Criteria=u2 > Threshold  Threshold=1/F  SaturateOnIntegerOverflow=off  InputSameDT=off
  RMS : Outport  VectorParamsAs1DForOutWhenUnconnected=off
  wires:
  Sqrt/1 -> Switch/1
  Switch/1 -> RMS/1
  Constant2/1 -> Data Type Conversion Inherited2/2
  Constant3/1 -> Data Type Conversion Inherited1/2
  Constant4/1 -> Integrator (Discrete or Continuous)1/2
  Data Type Conversion Inherited3/1 -> Switch/3
  Constant5/1 -> Data Type Conversion Inherited3/2
  Data Type Conversion Inherited2/1 -> Integrator (Discrete or Continuous)1/1
  Data Type Conversion Inherited1/1 -> Integrator (Discrete or Continuous)1/3
  Integrator (Discrete or Continuous)1/1 -> Switch/2
  Constant1/1 -> Data Type Conversion Inherited/2
  Data Type Conversion Inherited/1 -> Integrator (Discrete or Continuous)/3
  Periodic Difference (Discrete or Continuous)/1 -> Gain/1
  Gain/1 -> Sqrt/1
  Integrator (Discrete or Continuous)/1 -> Periodic Difference (Discrete or Continuous)/1
  u/1 -> Math Function/1, Data Type Conversion Inherited2/1, Data Type Conversion Inherited3/1, Data Type Conversion Inherited1/1
  Math Function/1 -> Integrator (Discrete or Continuous)/1, Data Type Conversion Inherited/1
  Constant/1 -> Integrator (Discrete or Continuous)/2

== system DWPT_fixed/RMS1/RMS Measurement/Harmonic RMS/SinCos ==
  u : Inport
  Data Type Conversion Inherited : sl_signal_attributes/Data Type Conversion Inherited  ConvertRealWorld=Real World Value  DoSatur=off
  Integrator with Wrapped State (Discrete or Continuous) : eeGeneralControl/Integrator with Wrapped State (Discrete or Continuous)  LabelModeActiveChoice=Continuous  WrappedStateUpperValue=2*pi  WrappedStateLowerValue=0  x0=0  Ts=Ts
  Mux : Mux  Inputs=2
  Radial frequencies : Constant  Value=2*pi*F*K
  sincos : Trigonometry  Operator=sincos
  SinCos : Outport  VectorParamsAs1DForOutWhenUnconnected=off
  wires:
  u/1 -> Data Type Conversion Inherited/1
  Radial frequencies/1 -> Data Type Conversion Inherited/2
  Data Type Conversion Inherited/1 -> Integrator with Wrapped State (Discrete or Continuous)/1
  Integrator with Wrapped State (Discrete or Continuous)/1 -> sincos/1
  Mux/1 -> SinCos/1
  sincos/1 -> Mux/1
  sincos/2 -> Mux/2

== system DWPT_fixed/RMS10/RMS Measurement/Harmonic RMS/SinCos ==
  u : Inport
  Data Type Conversion Inherited : sl_signal_attributes/Data Type Conversion Inherited  ConvertRealWorld=Real World Value  DoSatur=off
  Integrator with Wrapped State (Discrete or Continuous) : eeGeneralControl/Integrator with Wrapped State (Discrete or Continuous)  LabelModeActiveChoice=Continuous  WrappedStateUpperValue=2*pi  WrappedStateLowerValue=0  x0=0  Ts=Ts
  Mux : Mux  Inputs=2
  Radial frequencies : Constant  Value=2*pi*F*K
  sincos : Trigonometry  Operator=sincos
  SinCos : Outport  VectorParamsAs1DForOutWhenUnconnected=off
  wires:
  u/1 -> Data Type Conversion Inherited/1
  Radial frequencies/1 -> Data Type Conversion Inherited/2
  Data Type Conversion Inherited/1 -> Integrator with Wrapped State (Discrete or Continuous)/1
  Integrator with Wrapped State (Discrete or Continuous)/1 -> sincos/1
  Mux/1 -> SinCos/1
  sincos/1 -> Mux/1
  sincos/2 -> Mux/2

== system DWPT_fixed/RMS2/RMS Measurement/Harmonic RMS/SinCos ==
  u : Inport
  Data Type Conversion Inherited : sl_signal_attributes/Data Type Conversion Inherited  ConvertRealWorld=Real World Value  DoSatur=off
  Integrator with Wrapped State (Discrete or Continuous) : eeGeneralControl/Integrator with Wrapped State (Discrete or Continuous)  LabelModeActiveChoice=Continuous  WrappedStateUpperValue=2*pi  WrappedStateLowerValue=0  x0=0  Ts=Ts
  Mux : Mux  Inputs=2
  Radial frequencies : Constant  Value=2*pi*F*K
  sincos : Trigonometry  Operator=sincos
  SinCos : Outport  VectorParamsAs1DForOutWhenUnconnected=off
  wires:
  u/1 -> Data Type Conversion Inherited/1
  Radial frequencies/1 -> Data Type Conversion Inherited/2
  Data Type Conversion Inherited/1 -> Integrator with Wrapped State (Discrete or Continuous)/1
  Integrator with Wrapped State (Discrete or Continuous)/1 -> sincos/1
  Mux/1 -> SinCos/1
  sincos/1 -> Mux/1
  sincos/2 -> Mux/2

== system DWPT_fixed/RMS3/RMS Measurement/Harmonic RMS/SinCos ==
  u : Inport
  Data Type Conversion Inherited : sl_signal_attributes/Data Type Conversion Inherited  ConvertRealWorld=Real World Value  DoSatur=off
  Integrator with Wrapped State (Discrete or Continuous) : eeGeneralControl/Integrator with Wrapped State (Discrete or Continuous)  LabelModeActiveChoice=Continuous  WrappedStateUpperValue=2*pi  WrappedStateLowerValue=0  x0=0  Ts=Ts
  Mux : Mux  Inputs=2
  Radial frequencies : Constant  Value=2*pi*F*K
  sincos : Trigonometry  Operator=sincos
  SinCos : Outport  VectorParamsAs1DForOutWhenUnconnected=off
  wires:
  u/1 -> Data Type Conversion Inherited/1
  Radial frequencies/1 -> Data Type Conversion Inherited/2
  Data Type Conversion Inherited/1 -> Integrator with Wrapped State (Discrete or Continuous)/1
  Integrator with Wrapped State (Discrete or Continuous)/1 -> sincos/1
  Mux/1 -> SinCos/1
  sincos/1 -> Mux/1
  sincos/2 -> Mux/2

== system DWPT_fixed/RMS4/RMS Measurement/Harmonic RMS/SinCos ==
  u : Inport
  Data Type Conversion Inherited : sl_signal_attributes/Data Type Conversion Inherited  ConvertRealWorld=Real World Value  DoSatur=off
  Integrator with Wrapped State (Discrete or Continuous) : eeGeneralControl/Integrator with Wrapped State (Discrete or Continuous)  LabelModeActiveChoice=Continuous  WrappedStateUpperValue=2*pi  WrappedStateLowerValue=0  x0=0  Ts=Ts
  Mux : Mux  Inputs=2
  Radial frequencies : Constant  Value=2*pi*F*K
  sincos : Trigonometry  Operator=sincos
  SinCos : Outport  VectorParamsAs1DForOutWhenUnconnected=off
  wires:
  u/1 -> Data Type Conversion Inherited/1
  Radial frequencies/1 -> Data Type Conversion Inherited/2
  Data Type Conversion Inherited/1 -> Integrator with Wrapped State (Discrete or Continuous)/1
  Integrator with Wrapped State (Discrete or Continuous)/1 -> sincos/1
  Mux/1 -> SinCos/1
  sincos/1 -> Mux/1
  sincos/2 -> Mux/2

== system DWPT_fixed/RMS6/RMS Measurement/Harmonic RMS/SinCos ==
  u : Inport
  Data Type Conversion Inherited : sl_signal_attributes/Data Type Conversion Inherited  ConvertRealWorld=Real World Value  DoSatur=off
  Integrator with Wrapped State (Discrete or Continuous) : eeGeneralControl/Integrator with Wrapped State (Discrete or Continuous)  LabelModeActiveChoice=Continuous  WrappedStateUpperValue=2*pi  WrappedStateLowerValue=0  x0=0  Ts=Ts
  Mux : Mux  Inputs=2
  Radial frequencies : Constant  Value=2*pi*F*K
  sincos : Trigonometry  Operator=sincos
  SinCos : Outport  VectorParamsAs1DForOutWhenUnconnected=off
  wires:
  u/1 -> Data Type Conversion Inherited/1
  Radial frequencies/1 -> Data Type Conversion Inherited/2
  Data Type Conversion Inherited/1 -> Integrator with Wrapped State (Discrete or Continuous)/1
  Integrator with Wrapped State (Discrete or Continuous)/1 -> sincos/1
  Mux/1 -> SinCos/1
  sincos/1 -> Mux/1
  sincos/2 -> Mux/2

== system DWPT_fixed/RMS8/RMS Measurement/Harmonic RMS/SinCos ==
  u : Inport
  Data Type Conversion Inherited : sl_signal_attributes/Data Type Conversion Inherited  ConvertRealWorld=Real World Value  DoSatur=off
  Integrator with Wrapped State (Discrete or Continuous) : eeGeneralControl/Integrator with Wrapped State (Discrete or Continuous)  LabelModeActiveChoice=Continuous  WrappedStateUpperValue=2*pi  WrappedStateLowerValue=0  x0=0  Ts=Ts
  Mux : Mux  Inputs=2
  Radial frequencies : Constant  Value=2*pi*F*K
  sincos : Trigonometry  Operator=sincos
  SinCos : Outport  VectorParamsAs1DForOutWhenUnconnected=off
  wires:
  u/1 -> Data Type Conversion Inherited/1
  Radial frequencies/1 -> Data Type Conversion Inherited/2
  Data Type Conversion Inherited/1 -> Integrator with Wrapped State (Discrete or Continuous)/1
  Integrator with Wrapped State (Discrete or Continuous)/1 -> sincos/1
  Mux/1 -> SinCos/1
  sincos/1 -> Mux/1
  sincos/2 -> Mux/2
